simulink library "Linkage"  (R2025b)
settings: Solver=VariableStepAuto  StartTime=0.0  StopTime=10.0  RelTol=1e-3
undefined symbols (not defined in the file): Axle1D, AxleIn, Chassis, Init, RaceFix, RaceSpin, Vehicle, Visual, X, Y, Z
libraries: sm_lib x940, nesl_utility x136, fl_lib x6, Linkage_Systems x2, SteeringWheel x2, Linkage_Decoupled x2, AntiRollBar_Systems x1, Steer_Rack_None x1, Steer_Rack_WheelDrivenRack1UJoint x1
(part 15 of 25)

== system Linkage/Susp/Linkage Decoupled/Steer/Rack Driven Shafts/Driver/Human/Twist ==
  Revolute Joint : sm_lib/Joints/Revolute Joint  Commented=on  JointMode=Normal  CompositeWrenchDir=FollowerOnBase  CompositeWrenchFrame=BaseFrame  SenseConstraintForce=off  SenseConstraintTorque=off  SenseTotalForce=off  SenseTotalTorque=off  PositionTargetSpecify=off  PositionTargetPriority=High  PositionTargetValue=0  PositionTargetValueUnits=deg  VelocityTargetSpecify=off  VelocityTargetPriority=High  VelocityTargetValue=0  VelocityTargetValueUnits=deg/s  EquilibriumPosition=0  EquilibriumPositionUnits=deg  SpringStiffness=dt_k  SpringStiffnessUnits=N*m/deg  DampingCoefficient=dt_b  DampingCoefficientUnits=N*m/(deg/s)  LowerLimitSpecify=off  LowerLimitBound=-90  LowerLimitBoundUnits=deg  LowerLimitStiffness=1e4  LowerLimitStiffnessUnits=N*m/deg  LowerLimitDamping=10  LowerLimitDampingUnits=N*m/(deg/s)  LowerLimitTransitionRegionWidth=0.1  LowerLimitTransitionRegionWidthUnits=deg  UpperLimitSpecify=off  UpperLimitBound=90  UpperLimitBoundUnits=deg  UpperLimitStiffness=1e4  UpperLimitStiffnessUnits=N*m/deg  UpperLimitDamping=10  UpperLimitDampingUnits=N*m/(deg/s)  UpperLimitTransitionRegionWidth=0.1  UpperLimitTransitionRegionWidthUnits=deg  TorqueActuationMode=NoTorque  MotionActuationMode=ComputedMotion  SensePosition=off  SenseVelocity=off  SenseAcceleration=off  SenseTorqueForce=off  SenseLowerLimitTorqueForce=off  SenseUpperLimitTorqueForce=off
  Transform Axis Location B : sm_lib/Frames and Transforms/Rigid Transform  RotationMethod=None  FollAlignAxisA=+X  BaseAlignAxisA=+Y  FollAlignAxisB=+Y  BaseAlignAxisB=+Z  RotationStandardAxis=+Y  RotationAngle=0  RotationAngleUnits=deg  RotationArbitraryAxis=[0 0 1]  RotationSequenceAxes=FollowerAxes  RotationSequence=XYX  RotationSequenceAngles=[0 0 0]  RotationSequenceAnglesUnits=deg  RotationMatrix=[1 0 0; 0 1 0; 0 0 1]  Quaternion=[1 0 0 0]  TranslationMethod=StandardAxis  TranslationCartesianOffset=[0 0 0]  TranslationCartesianOffsetUnits=m  TranslationStandardAxis=-X  TranslationStandardOffset=0.05  TranslationStandardOffsetUnits=m  TranslationROffset=0  TranslationROffsetUnits=m  TranslationThetaOffset=0  TranslationThetaOffsetUnits=deg  TranslationZOffset=0  TranslationZOffsetUnits=m
  Transform Axis Location F : sm_lib/Frames and Transforms/Rigid Transform  RotationMethod=None  FollAlignAxisA=+X  BaseAlignAxisA=+Y  FollAlignAxisB=+Y  BaseAlignAxisB=+Z  RotationStandardAxis=+Y  RotationAngle=0  RotationAngleUnits=deg  RotationArbitraryAxis=[0 0 1]  RotationSequenceAxes=FollowerAxes  RotationSequence=XYX  RotationSequenceAngles=[0 0 0]  RotationSequenceAnglesUnits=deg  RotationMatrix=[1 0 0; 0 1 0; 0 0 1]  Quaternion=[1 0 0 0]  TranslationMethod=StandardAxis  TranslationCartesianOffset=[0 0 0]  TranslationCartesianOffsetUnits=m  TranslationStandardAxis=-X  TranslationStandardOffset=0.05  TranslationStandardOffsetUnits=m  TranslationROffset=0  TranslationROffsetUnits=m  TranslationThetaOffset=0  TranslationThetaOffsetUnits=deg  TranslationZOffset=0  TranslationZOffsetUnits=m
  Transform Axis Orientation B : sm_lib/Frames and Transforms/Rigid Transform  RotationMethod=StandardAxis  FollAlignAxisA=+X  BaseAlignAxisA=+Y  FollAlignAxisB=+Y  BaseAlignAxisB=+Z  RotationStandardAxis=+Y  RotationAngle=120  RotationAngleUnits=deg  RotationArbitraryAxis=[0 0 1]  RotationSequenceAxes=FollowerAxes  RotationSequence=XYX  RotationSequenceAngles=[0 0 0]  RotationSequenceAnglesUnits=deg  RotationMatrix=[1 0 0; 0 1 0; 0 0 1]  Quaternion=[1 0 0 0]  TranslationMethod=None  TranslationCartesianOffset=[0 0 0]  TranslationCartesianOffsetUnits=m  TranslationStandardAxis=+Z  TranslationStandardOffset=0  TranslationStandardOffsetUnits=m  TranslationROffset=0  TranslationROffsetUnits=m  TranslationThetaOffset=0  TranslationThetaOffsetUnits=deg  TranslationZOffset=0  TranslationZOffsetUnits=m
  Transform Axis Orientation F : sm_lib/Frames and Transforms/Rigid Transform  RotationMethod=StandardAxis  FollAlignAxisA=+X  BaseAlignAxisA=+Y  FollAlignAxisB=+Y  BaseAlignAxisB=+Z  RotationStandardAxis=+Y  RotationAngle=120  RotationAngleUnits=deg  RotationArbitraryAxis=[0 0 1]  RotationSequenceAxes=FollowerAxes  RotationSequence=XYX  RotationSequenceAngles=[0 0 0]  RotationSequenceAnglesUnits=deg  RotationMatrix=[1 0 0; 0 1 0; 0 0 1]  Quaternion=[1 0 0 0]  TranslationMethod=None  TranslationCartesianOffset=[0 0 0]  TranslationCartesianOffsetUnits=m  TranslationStandardAxis=+Z  TranslationStandardOffset=0  TranslationStandardOffsetUnits=m  TranslationROffset=0  TranslationROffsetUnits=m  TranslationThetaOffset=0  TranslationThetaOffsetUnits=deg  TranslationZOffset=0  TranslationZOffsetUnits=m
  Transform Universal B : sm_lib/Frames and Transforms/Rigid Transform  RotationMethod=StandardAxis  FollAlignAxisA=+X  BaseAlignAxisA=+Y  FollAlignAxisB=+Y  BaseAlignAxisB=+Z  RotationStandardAxis=+Y  RotationAngle=90  RotationAngleUnits=deg  RotationArbitraryAxis=[0 0 1]  RotationSequenceAxes=FollowerAxes  RotationSequence=XYX  RotationSequenceAngles=[0 0 0]  RotationSequenceAnglesUnits=deg  RotationMatrix=[1 0 0; 0 1 0; 0 0 1]  Quaternion=[1 0 0 0]  TranslationMethod=None  TranslationCartesianOffset=[0 0 0]  TranslationCartesianOffsetUnits=m  TranslationStandardAxis=+Z  TranslationStandardOffset=0  TranslationStandardOffsetUnits=m  TranslationROffset=0  TranslationROffsetUnits=m  TranslationThetaOffset=0  TranslationThetaOffsetUnits=deg  TranslationZOffset=0  TranslationZOffsetUnits=m
  Transform Universal F : sm_lib/Frames and Transforms/Rigid Transform  RotationMethod=StandardAxis  FollAlignAxisA=+X  BaseAlignAxisA=+Y  FollAlignAxisB=+Y  BaseAlignAxisB=+Z  RotationStandardAxis=+Y  RotationAngle=90  RotationAngleUnits=deg  RotationArbitraryAxis=[0 0 1]  RotationSequenceAxes=FollowerAxes  RotationSequence=XYX  RotationSequenceAngles=[0 0 0]  RotationSequenceAnglesUnits=deg  RotationMatrix=[1 0 0; 0 1 0; 0 0 1]  Quaternion=[1 0 0 0]  TranslationMethod=None  TranslationCartesianOffset=[0 0 0]  TranslationCartesianOffsetUnits=m  TranslationStandardAxis=+Z  TranslationStandardOffset=0  TranslationStandardOffsetUnits=m  TranslationROffset=0  TranslationROffsetUnits=m  TranslationThetaOffset=0  TranslationThetaOffsetUnits=deg  TranslationZOffset=0  TranslationZOffsetUnits=m
  Universal Torso : sm_lib/Joints/Universal Joint  JointMode=Normal  CompositeWrenchDir=FollowerOnBase  CompositeWrenchFrame=BaseFrame  SenseConstraintForce=off  SenseConstraintTorque=off  SenseTotalForce=off  SenseTotalTorque=off  RxPositionTargetSpecify=off  RxPositionTargetPriority=High  RxPositionTargetValue=0  RxPositionTargetValueUnits=deg  RxVelocityTargetSpecify=off  RxVelocityTargetPriority=High  RxVelocityTargetValue=0  RxVelocityTargetValueUnits=deg/s  RxEquilibriumPosition=0  RxEquilibriumPositionUnits=deg  RxSpringStiffness=10  RxSpringStiffnessUnits=N*m/deg  RxDampingCoefficient=1  RxDampingCoefficientUnits=N*m/(deg/s)  RxLowerLimitSpecify=off  RxLowerLimitBound=-90  RxLowerLimitBoundUnits=deg  RxLowerLimitStiffness=1e4  RxLowerLimitStiffnessUnits=N*m/deg  RxLowerLimitDamping=10  RxLowerLimitDampingUnits=N*m/(deg/s)  RxLowerLimitTransitionRegionWidth=0.1  RxLowerLimitTransitionRegionWidthUnits=deg  RxUpperLimitSpecify=off  RxUpperLimitBound=90  RxUpperLimitBoundUnits=deg  RxUpperLimitStiffness=1e4  RxUpperLimitStiffnessUnits=N*m/deg  RxUpperLimitDamping=10  RxUpperLimitDampingUnits=N*m/(deg/s)  RxUpperLimitTransitionRegionWidth=0.1  RxUpperLimitTransitionRegionWidthUnits=deg  RxTorqueActuationMode=NoTorque  RxMotionActuationMode=ComputedMotion  RxSensePosition=off  RxSenseVelocity=off  RxSenseAcceleration=off  RxSenseTorqueForce=off  RxSenseLowerLimitTorqueForce=off  RxSenseUpperLimitTorqueForce=off  RyPositionTargetSpecify=off  RyPositionTargetPriority=High  RyPositionTargetValue=0  RyPositionTargetValueUnits=deg  RyVelocityTargetSpecify=off  RyVelocityTargetPriority=High  RyVelocityTargetValue=0  RyVelocityTargetValueUnits=deg/s  RyEquilibriumPosition=0  RyEquilibriumPositionUnits=deg  RySpringStiffness=10  RySpringStiffnessUnits=N*m/deg  RyDampingCoefficient=1  RyDampingCoefficientUnits=N*m/(deg/s)  RyLowerLimitSpecify=off  RyLowerLimitBound=-90  RyLowerLimitBoundUnits=deg  RyLowerLimitStiffness=1e4  RyLowerLimitStiffnessUnits=N*m/deg  RyLowerLimitDamping=10  RyLowerLimitDampingUnits=N*m/(deg/s)  RyLowerLimitTransitionRegionWidth=0.1  RyLowerLimitTransitionRegionWidthUnits=deg  RyUpperLimitSpecify=off  RyUpperLimitBound=90  RyUpperLimitBoundUnits=deg  RyUpperLimitStiffness=1e4  RyUpperLimitStiffnessUnits=N*m/deg  RyUpperLimitDamping=10  RyUpperLimitDampingUnits=N*m/(deg/s)  RyUpperLimitTransitionRegionWidth=0.1  RyUpperLimitTransitionRegionWidthUnits=deg  RyTorqueActuationMode=NoTorque  RyMotionActuationMode=ComputedMotion  RySensePosition=off  RySenseVelocity=off  RySenseAcceleration=off  RySenseTorqueForce=off  RySenseLowerLimitTorqueForce=off  RySenseUpperLimitTorqueForce=off
  T : PMIOPort  Side=Right
  B : PMIOPort  Port=2  Side=Left
  connections:
  Transform Axis Orientation B/RConn1 -- Transform Axis Location B/LConn1
  B/RConn1 -- Transform Axis Orientation B/LConn1
  Transform Axis Orientation F/RConn1 -- Transform Axis Location F/LConn1
  Transform Axis Location B/RConn1 -- Transform Universal B/LConn1
  Transform Axis Orientation F/LConn1 -- T/RConn1
  Transform Axis Location F/RConn1 -- Transform Universal F/LConn1
  Universal Torso/LConn1 -- Transform Universal B/RConn1
  Universal Torso/RConn1 -- Transform Universal F/RConn1

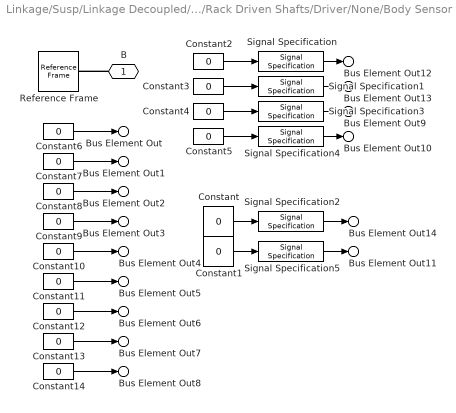
== system Linkage/Susp/Linkage Decoupled/Steer/Rack Driven Shafts/Driver/None/Body Sensor Empty ==
  Constant{,1..14} (15 alike) : Constant  Value=0
  Reference Frame : sm_lib/Frames and Transforms/Reference Frame
  Signal Specification : SignalSpecification  Unit=rad
  Signal Specification1 : SignalSpecification  Unit=rad
  Signal Specification2 : SignalSpecification  Unit=rad
  Signal Specification3 : SignalSpecification  Unit=rad/s
  Signal Specification4 : SignalSpecification  Unit=rad/s
  Signal Specification5 : SignalSpecification  Unit=rad/s
  B : PMIOPort  Side=Left
  Bus Element Out : Outport  VectorParamsAs1DForOutWhenUnconnected=off  PortName=Body  Element=x
  Bus Element Out1 : Outport  VectorParamsAs1DForOutWhenUnconnected=off  PortName=Body  Element=y
  Bus Element Out2 : Outport  VectorParamsAs1DForOutWhenUnconnected=off  PortName=Body  Element=z
  Bus Element Out3 : Outport  VectorParamsAs1DForOutWhenUnconnected=off  PortName=Body  Element=vx
  Bus Element Out4 : Outport  VectorParamsAs1DForOutWhenUnconnected=off  PortName=Body  Element=vy
  Bus Element Out5 : Outport  VectorParamsAs1DForOutWhenUnconnected=off  PortName=Body  Element=vz
  Bus Element Out6 : Outport  VectorParamsAs1DForOutWhenUnconnected=off  PortName=Body  Element=gx
  Bus Element Out7 : Outport  VectorParamsAs1DForOutWhenUnconnected=off  PortName=Body  Element=gy
  Bus Element Out8 : Outport  VectorParamsAs1DForOutWhenUnconnected=off  PortName=Body  Element=gz
  Bus Element Out9 : Outport  VectorParamsAs1DForOutWhenUnconnected=off  PortName=Body  Element=nRoll
  Bus Element Out10 : Outport  VectorParamsAs1DForOutWhenUnconnected=off  PortName=Body  Element=nPitch
  Bus Element Out11 : Outport  VectorParamsAs1DForOutWhenUnconnected=off  PortName=Body  Element=nYaw
  Bus Element Out12 : Outport  VectorParamsAs1DForOutWhenUnconnected=off  PortName=Body  Element=aRoll
  Bus Element Out13 : Outport  VectorParamsAs1DForOutWhenUnconnected=off  PortName=Body  Element=aPitch
  Bus Element Out14 : Outport  VectorParamsAs1DForOutWhenUnconnected=off  PortName=Body  Element=aYaw
  wires:
  Constant14/1 -> Bus Element Out8/1
  Constant11/1 -> Bus Element Out5/1
  Constant12/1 -> Bus Element Out6/1
  Constant7/1 -> Bus Element Out1/1
  Constant13/1 -> Bus Element Out7/1
  Constant10/1 -> Bus Element Out4/1
  Constant8/1 -> Bus Element Out2/1
  Constant6/1 -> Bus Element Out/1
  Constant9/1 -> Bus Element Out3/1
  Signal Specification/1 -> Bus Element Out12/1
  Signal Specification1/1 -> Bus Element Out13/1
  Signal Specification2/1 -> Bus Element Out14/1
  Signal Specification3/1 -> Bus Element Out9/1
  Signal Specification4/1 -> Bus Element Out10/1
  Signal Specification5/1 -> Bus Element Out11/1
  Constant/1 -> Signal Specification2/1
  Constant1/1 -> Signal Specification5/1
  Constant4/1 -> Signal Specification3/1
  Constant5/1 -> Signal Specification4/1
  Constant3/1 -> Signal Specification1/1
  Constant2/1 -> Signal Specification/1
  connections:
  B/RConn1 -- Reference Frame/RConn1

== system Linkage/Susp/Linkage Decoupled/Steer/Rack Driven Shafts/Wheel/FSAE/Transform Steer Axis ==
  Rigid Transform1 : sm_lib/Frames and Transforms/Rigid Transform  RotationMethod=None  FollAlignAxisA=+X  BaseAlignAxisA=+Y  FollAlignAxisB=+Y  BaseAlignAxisB=+Z  RotationStandardAxis=+Z  RotationAngle=0.0  RotationAngleUnits=deg  RotationArbitraryAxis=[0 0 1]  RotationSequenceAxes=FollowerAxes  RotationSequence=XYX  RotationSequenceAngles=[0 0 0]  RotationSequenceAnglesUnits=deg  RotationMatrix=[1 0 0; 0 1 0; 0 0 1]  Quaternion=[1 0 0 0]  TranslationMethod=Cartesian  TranslationCartesianOffset=[0 -0.4664 -0.3791]  TranslationCartesianOffsetUnits=m  TranslationStandardAxis=+Z  TranslationStandardOffset=0  TranslationStandardOffsetUnits=m  TranslationROffset=0  TranslationROffsetUnits=m  TranslationThetaOffset=0  TranslationThetaOffsetUnits=deg  TranslationZOffset=0  TranslationZOffsetUnits=m
  Rigid Transform2 : sm_lib/Frames and Transforms/Rigid Transform  RotationMethod=RotationMatrix  FollAlignAxisA=+X  BaseAlignAxisA=+Y  FollAlignAxisB=+Y  BaseAlignAxisB=+Z  RotationStandardAxis=+Z  RotationAngle=0.0  RotationAngleUnits=deg  RotationArbitraryAxis=[0 0 1]  RotationSequenceAxes=FollowerAxes  RotationSequence=XYX  RotationSequenceAngles=[0 0 0]  RotationSequenceAnglesUnits=deg  RotationMatrix=[0.5 0.866 -6.661e-16; -0.8602 0.4967 0.1153; 0.09988 -0.05766 0.9933]  Quaternion=[1 0 0 0]  TranslationMethod=None  TranslationCartesianOffset=[0 0 0]  TranslationCartesianOffsetUnits=m  TranslationStandardAxis=+Z  TranslationStandardOffset=0  TranslationStandardOffsetUnits=m  TranslationROffset=0  TranslationROffsetUnits=m  TranslationThetaOffset=0  TranslationThetaOffsetUnits=deg  TranslationZOffset=0  TranslationZOffsetUnits=m
  Rigid Transform4 : sm_lib/Frames and Transforms/Rigid Transform  RotationMethod=StandardAxis  FollAlignAxisA=+X  BaseAlignAxisA=+Y  FollAlignAxisB=+Y  BaseAlignAxisB=+Z  RotationStandardAxis=+Z  RotationAngle=150  RotationAngleUnits=deg  RotationArbitraryAxis=[0 0 1]  RotationSequenceAxes=FollowerAxes  RotationSequence=XYX  RotationSequenceAngles=[0 0 0]  RotationSequenceAnglesUnits=deg  RotationMatrix=[1 0 0; 0 1 0; 0 0 1]  Quaternion=[1 0 0 0]  TranslationMethod=StandardAxis  TranslationCartesianOffset=[0 0 0]  TranslationCartesianOffsetUnits=m  TranslationStandardAxis=+Z  TranslationStandardOffset=0.09  TranslationStandardOffsetUnits=m  TranslationROffset=0  TranslationROffsetUnits=m  TranslationThetaOffset=0  TranslationThetaOffsetUnits=deg  TranslationZOffset=0  TranslationZOffsetUnits=m
  F : PMIOPort  Side=Left
  B : PMIOPort  Port=2  Side=Right
  connections:
  Rigid Transform2/RConn1 -- Rigid Transform4/LConn1
  F/RConn1 -- Rigid Transform4/RConn1
  Rigid Transform1/LConn1 -- Rigid Transform2/LConn1
  B/RConn1 -- Rigid Transform1/RConn1

== system Linkage/Susp/Linkage Decoupled/Steer/Rack Static Shafts/Driver/Human/Arm L ==
  Arm Lower L : Subsystem
  Arm Upper L : Subsystem
  Hand L : Subsystem
  Revolute ElbowL : sm_lib/Joints/Revolute Joint  JointMode=Normal  CompositeWrenchDir=FollowerOnBase  CompositeWrenchFrame=BaseFrame  SenseConstraintForce=off  SenseConstraintTorque=off  SenseTotalForce=off  SenseTotalTorque=off  PositionTargetSpecify=on  PositionTargetPriority=Low  PositionTargetValue=50  PositionTargetValueUnits=deg  VelocityTargetSpecify=off  VelocityTargetPriority=High  VelocityTargetValue=0  VelocityTargetValueUnits=deg/s  EquilibriumPosition=0  EquilibriumPositionUnits=deg  SpringStiffness=0  SpringStiffnessUnits=N*m/deg  DampingCoefficient=0  DampingCoefficientUnits=N*m/(deg/s)  LowerLimitSpecify=off  LowerLimitBound=-90  LowerLimitBoundUnits=deg  LowerLimitStiffness=1e4  LowerLimitStiffnessUnits=N*m/deg  LowerLimitDamping=10  LowerLimitDampingUnits=N*m/(deg/s)  LowerLimitTransitionRegionWidth=0.1  LowerLimitTransitionRegionWidthUnits=deg  UpperLimitSpecify=off  UpperLimitBound=90  UpperLimitBoundUnits=deg  UpperLimitStiffness=1e4  UpperLimitStiffnessUnits=N*m/deg  UpperLimitDamping=10  UpperLimitDampingUnits=N*m/(deg/s)  UpperLimitTransitionRegionWidth=0.1  UpperLimitTransitionRegionWidthUnits=deg  TorqueActuationMode=NoTorque  MotionActuationMode=ComputedMotion  SensePosition=off  SenseVelocity=off  SenseAcceleration=off  SenseTorqueForce=off  SenseLowerLimitTorqueForce=off  SenseUpperLimitTorqueForce=off
  Spherical ShoulderL : sm_lib/Joints/Spherical Joint  JointMode=Normal  CompositeWrenchDir=FollowerOnBase  CompositeWrenchFrame=BaseFrame  SenseConstraintForce=off  SenseConstraintTorque=off  SenseTotalForce=off  SenseTotalTorque=off  PositionTargetSpecify=off  PositionTargetPriority=High  PositionTargetRotationMethod=None  PositionTargetFollAlignAxisA=+X  PositionTargetBaseAlignAxisA=+Y  PositionTargetFollAlignAxisB=+Y  PositionTargetBaseAlignAxisB=+Z  PositionTargetRotationStandardAxis=+Z  PositionTargetRotationAngle=0.0  PositionTargetRotationAngleUnits=deg  PositionTargetRotationArbitraryAxis=[0 0 1]  PositionTargetRotationSequenceAxes=FollowerAxes  PositionTargetRotationSequence=XYX  PositionTargetRotationSequenceAngles=[0 0 0]  PositionTargetRotationSequenceAnglesUnits=deg  PositionTargetRotationMatrix=[1 0 0; 0 1 0; 0 0 1]  PositionTargetQuaternion=[1 0 0 0]  VelocityTargetSpecify=off  VelocityTargetPriority=High  VelocityTargetValue=[0 0 0]  VelocityTargetValueUnits=deg/s  VelocityTargetInFollowerFrame=on  EqPosRotationMethod=None  EqPosFollAlignAxisA=+X  EqPosBaseAlignAxisA=+Y  EqPosFollAlignAxisB=+Y  EqPosBaseAlignAxisB=+Z  EqPosRotationStandardAxis=+Z  EqPosRotationAngle=0.0  EqPosRotationAngleUnits=deg  EqPosRotationArbitraryAxis=[0 0 1]  EqPosRotationSequenceAxes=FollowerAxes  EqPosRotationSequence=XYX  EqPosRotationSequenceAngles=[0 0 0]  EqPosRotationSequenceAnglesUnits=deg  EqPosRotationMatrix=[1 0 0; 0 1 0; 0 0 1]  EqPosQuaternion=[1 0 0 0]  SpringStiffness=0  SpringStiffnessUnits=N*m/deg  DampingCoefficient=0  DampingCoefficientUnits=N*m/(deg/s)  LowerLimitSpecify=off  LowerLimitBound=15  LowerLimitBoundUnits=deg  LowerLimitStiffness=1e4  LowerLimitStiffnessUnits=N*m/deg  LowerLimitDamping=10  LowerLimitDampingUnits=N*m/(deg/s)  LowerLimitTransitionRegionWidth=0.1  LowerLimitTransitionRegionWidthUnits=deg  UpperLimitSpecify=off  UpperLimitBound=45  UpperLimitBoundUnits=deg  UpperLimitStiffness=1e4  UpperLimitStiffnessUnits=N*m/deg  UpperLimitDamping=10  UpperLimitDampingUnits=N*m/(deg/s)  UpperLimitTransitionRegionWidth=0.1  UpperLimitTransitionRegionWidthUnits=deg  TorqueActuationMode=NoTorque  ActuateTorqueX=off  ActuateTorqueY=off  ActuateTorqueZ=off  ActuateTorque=off  ActuationFrame=BaseFrame  SensePosition=off  SenseVelocityX=off  SenseVelocityY=off  SenseVelocityZ=off  SenseVelocity=off  SenseAccelerationX=off  SenseAccelerationY=off  SenseAccelerationZ=off  SenseAcceleration=off  SenseLowerLimitTorqueMag=off  SenseUpperLimitTorqueMag=off  SensingFrame=BaseFrame
  Universal WristL : sm_lib/Joints/Universal Joint  JointMode=Normal  CompositeWrenchDir=FollowerOnBase  CompositeWrenchFrame=BaseFrame  SenseConstraintForce=off  SenseConstraintTorque=off  SenseTotalForce=off  SenseTotalTorque=off  RxPositionTargetSpecify=off  RxPositionTargetPriority=High  RxPositionTargetValue=0  RxPositionTargetValueUnits=deg  RxVelocityTargetSpecify=off  RxVelocityTargetPriority=High  RxVelocityTargetValue=0  RxVelocityTargetValueUnits=deg/s  RxEquilibriumPosition=0  RxEquilibriumPositionUnits=deg  RxSpringStiffness=0  RxSpringStiffnessUnits=N*m/deg  RxDampingCoefficient=0  RxDampingCoefficientUnits=N*m/(deg/s)  RxLowerLimitSpecify=off  RxLowerLimitBound=-90  RxLowerLimitBoundUnits=deg  RxLowerLimitStiffness=1e4  RxLowerLimitStiffnessUnits=N*m/deg  RxLowerLimitDamping=10  RxLowerLimitDampingUnits=N*m/(deg/s)  RxLowerLimitTransitionRegionWidth=0.1  RxLowerLimitTransitionRegionWidthUnits=deg  RxUpperLimitSpecify=off  RxUpperLimitBound=90  RxUpperLimitBoundUnits=deg  RxUpperLimitStiffness=1e4  RxUpperLimitStiffnessUnits=N*m/deg  RxUpperLimitDamping=10  RxUpperLimitDampingUnits=N*m/(deg/s)  RxUpperLimitTransitionRegionWidth=0.1  RxUpperLimitTransitionRegionWidthUnits=deg  RxTorqueActuationMode=NoTorque  RxMotionActuationMode=ComputedMotion  RxSensePosition=off  RxSenseVelocity=off  RxSenseAcceleration=off  RxSenseTorqueForce=off  RxSenseLowerLimitTorqueForce=off  RxSenseUpperLimitTorqueForce=off  RyPositionTargetSpecify=off  RyPositionTargetPriority=High  RyPositionTargetValue=0  RyPositionTargetValueUnits=deg  RyVelocityTargetSpecify=off  RyVelocityTargetPriority=High  RyVelocityTargetValue=0  RyVelocityTargetValueUnits=deg/s  RyEquilibriumPosition=0  RyEquilibriumPositionUnits=deg  RySpringStiffness=0  RySpringStiffnessUnits=N*m/deg  RyDampingCoefficient=0  RyDampingCoefficientUnits=N*m/(deg/s)  RyLowerLimitSpecify=off  RyLowerLimitBound=-90  RyLowerLimitBoundUnits=deg  RyLowerLimitStiffness=1e4  RyLowerLimitStiffnessUnits=N*m/deg  RyLowerLimitDamping=10  RyLowerLimitDampingUnits=N*m/(deg/s)  RyLowerLimitTransitionRegionWidth=0.1  RyLowerLimitTransitionRegionWidthUnits=deg  RyUpperLimitSpecify=off  RyUpperLimitBound=90  RyUpperLimitBoundUnits=deg  RyUpperLimitStiffness=1e4  RyUpperLimitStiffnessUnits=N*m/deg  RyUpperLimitDamping=10  RyUpperLimitDampingUnits=N*m/(deg/s)  RyUpperLimitTransitionRegionWidth=0.1  RyUpperLimitTransitionRegionWidthUnits=deg  RyTorqueActuationMode=NoTorque  RyMotionActuationMode=ComputedMotion  RySensePosition=off  RySenseVelocity=off  RySenseAcceleration=off  RySenseTorqueForce=off  RySenseLowerLimitTorqueForce=off  RySenseUpperLimitTorqueForce=off
  Sh : PMIOPort  Side=Left
  Grip : PMIOPort  Port=2  Side=Right
  connections:
  Spherical ShoulderL/LConn1 -- Sh/RConn1
  Arm Lower L/RConn1 -- Universal WristL/LConn1
  Arm Lower L/LConn1 -- Revolute ElbowL/RConn1
  Hand L/RConn1 -- Grip/RConn1
  Universal WristL/RConn1 -- Hand L/LConn1
  Spherical ShoulderL/RConn1 -- Arm Upper L/LConn1
  Revolute ElbowL/LConn1 -- Arm Upper L/RConn1

== system Linkage/Susp/Linkage Decoupled/Steer/Rack Static Shafts/Driver/Human/Arm R ==
  Arm Lower R : Subsystem
  Arm Upper R : Subsystem
  Hand R : Subsystem
  Revolute ElbowR : sm_lib/Joints/Revolute Joint  JointMode=Normal  CompositeWrenchDir=FollowerOnBase  CompositeWrenchFrame=BaseFrame  SenseConstraintForce=off  SenseConstraintTorque=off  SenseTotalForce=off  SenseTotalTorque=off  PositionTargetSpecify=on  PositionTargetPriority=Low  PositionTargetValue=50  PositionTargetValueUnits=deg  VelocityTargetSpecify=off  VelocityTargetPriority=High  VelocityTargetValue=0  VelocityTargetValueUnits=deg/s  EquilibriumPosition=0  EquilibriumPositionUnits=deg  SpringStiffness=0  SpringStiffnessUnits=N*m/deg  DampingCoefficient=0  DampingCoefficientUnits=N*m/(deg/s)  LowerLimitSpecify=off  LowerLimitBound=-90  LowerLimitBoundUnits=deg  LowerLimitStiffness=1e4  LowerLimitStiffnessUnits=N*m/deg  LowerLimitDamping=10  LowerLimitDampingUnits=N*m/(deg/s)  LowerLimitTransitionRegionWidth=0.1  LowerLimitTransitionRegionWidthUnits=deg  UpperLimitSpecify=off  UpperLimitBound=90  UpperLimitBoundUnits=deg  UpperLimitStiffness=1e4  UpperLimitStiffnessUnits=N*m/deg  UpperLimitDamping=10  UpperLimitDampingUnits=N*m/(deg/s)  UpperLimitTransitionRegionWidth=0.1  UpperLimitTransitionRegionWidthUnits=deg  TorqueActuationMode=NoTorque  MotionActuationMode=ComputedMotion  SensePosition=off  SenseVelocity=off  SenseAcceleration=off  SenseTorqueForce=off  SenseLowerLimitTorqueForce=off  SenseUpperLimitTorqueForce=off
  Spherical ShoulderR : sm_lib/Joints/Spherical Joint  JointMode=Normal  CompositeWrenchDir=FollowerOnBase  CompositeWrenchFrame=BaseFrame  SenseConstraintForce=off  SenseConstraintTorque=off  SenseTotalForce=off  SenseTotalTorque=off  PositionTargetSpecify=off  PositionTargetPriority=High  PositionTargetRotationMethod=None  PositionTargetFollAlignAxisA=+X  PositionTargetBaseAlignAxisA=+Y  PositionTargetFollAlignAxisB=+Y  PositionTargetBaseAlignAxisB=+Z  PositionTargetRotationStandardAxis=+Z  PositionTargetRotationAngle=0.0  PositionTargetRotationAngleUnits=deg  PositionTargetRotationArbitraryAxis=[0 0 1]  PositionTargetRotationSequenceAxes=FollowerAxes  PositionTargetRotationSequence=XYX  PositionTargetRotationSequenceAngles=[0 0 0]  PositionTargetRotationSequenceAnglesUnits=deg  PositionTargetRotationMatrix=[1 0 0; 0 1 0; 0 0 1]  PositionTargetQuaternion=[1 0 0 0]  VelocityTargetSpecify=off  VelocityTargetPriority=High  VelocityTargetValue=[0 0 0]  VelocityTargetValueUnits=deg/s  VelocityTargetInFollowerFrame=on  EqPosRotationMethod=None  EqPosFollAlignAxisA=+X  EqPosBaseAlignAxisA=+Y  EqPosFollAlignAxisB=+Y  EqPosBaseAlignAxisB=+Z  EqPosRotationStandardAxis=+Z  EqPosRotationAngle=0.0  EqPosRotationAngleUnits=deg  EqPosRotationArbitraryAxis=[0 0 1]  EqPosRotationSequenceAxes=FollowerAxes  EqPosRotationSequence=XYX  EqPosRotationSequenceAngles=[0 0 0]  EqPosRotationSequenceAnglesUnits=deg  EqPosRotationMatrix=[1 0 0; 0 1 0; 0 0 1]  EqPosQuaternion=[1 0 0 0]  SpringStiffness=0  SpringStiffnessUnits=N*m/deg  DampingCoefficient=0  DampingCoefficientUnits=N*m/(deg/s)  LowerLimitSpecify=off  LowerLimitBound=15  LowerLimitBoundUnits=deg  LowerLimitStiffness=1e4  LowerLimitStiffnessUnits=N*m/deg  LowerLimitDamping=10  LowerLimitDampingUnits=N*m/(deg/s)  LowerLimitTransitionRegionWidth=0.1  LowerLimitTransitionRegionWidthUnits=deg  UpperLimitSpecify=off  UpperLimitBound=45  UpperLimitBoundUnits=deg  UpperLimitStiffness=1e4  UpperLimitStiffnessUnits=N*m/deg  UpperLimitDamping=10  UpperLimitDampingUnits=N*m/(deg/s)  UpperLimitTransitionRegionWidth=0.1  UpperLimitTransitionRegionWidthUnits=deg  TorqueActuationMode=NoTorque  ActuateTorqueX=off  ActuateTorqueY=off  ActuateTorqueZ=off  ActuateTorque=off  ActuationFrame=BaseFrame  SensePosition=off  SenseVelocityX=off  SenseVelocityY=off  SenseVelocityZ=off  SenseVelocity=off  SenseAccelerationX=off  SenseAccelerationY=off  SenseAccelerationZ=off  SenseAcceleration=off  SenseLowerLimitTorqueMag=off  SenseUpperLimitTorqueMag=off  SensingFrame=BaseFrame
  Universal WristR : sm_lib/Joints/Universal Joint  JointMode=Normal  CompositeWrenchDir=FollowerOnBase  CompositeWrenchFrame=BaseFrame  SenseConstraintForce=off  SenseConstraintTorque=off  SenseTotalForce=off  SenseTotalTorque=off  RxPositionTargetSpecify=off  RxPositionTargetPriority=High  RxPositionTargetValue=0  RxPositionTargetValueUnits=deg  RxVelocityTargetSpecify=off  RxVelocityTargetPriority=High  RxVelocityTargetValue=0  RxVelocityTargetValueUnits=deg/s  RxEquilibriumPosition=0  RxEquilibriumPositionUnits=deg  RxSpringStiffness=0  RxSpringStiffnessUnits=N*m/deg  RxDampingCoefficient=0  RxDampingCoefficientUnits=N*m/(deg/s)  RxLowerLimitSpecify=off  RxLowerLimitBound=-90  RxLowerLimitBoundUnits=deg  RxLowerLimitStiffness=1e4  RxLowerLimitStiffnessUnits=N*m/deg  RxLowerLimitDamping=10  RxLowerLimitDampingUnits=N*m/(deg/s)  RxLowerLimitTransitionRegionWidth=0.1  RxLowerLimitTransitionRegionWidthUnits=deg  RxUpperLimitSpecify=off  RxUpperLimitBound=90  RxUpperLimitBoundUnits=deg  RxUpperLimitStiffness=1e4  RxUpperLimitStiffnessUnits=N*m/deg  RxUpperLimitDamping=10  RxUpperLimitDampingUnits=N*m/(deg/s)  RxUpperLimitTransitionRegionWidth=0.1  RxUpperLimitTransitionRegionWidthUnits=deg  RxTorqueActuationMode=NoTorque  RxMotionActuationMode=ComputedMotion  RxSensePosition=off  RxSenseVelocity=off  RxSenseAcceleration=off  RxSenseTorqueForce=off  RxSenseLowerLimitTorqueForce=off  RxSenseUpperLimitTorqueForce=off  RyPositionTargetSpecify=off  RyPositionTargetPriority=High  RyPositionTargetValue=0  RyPositionTargetValueUnits=deg  RyVelocityTargetSpecify=off  RyVelocityTargetPriority=High  RyVelocityTargetValue=0  RyVelocityTargetValueUnits=deg/s  RyEquilibriumPosition=0  RyEquilibriumPositionUnits=deg  RySpringStiffness=0  RySpringStiffnessUnits=N*m/deg  RyDampingCoefficient=0  RyDampingCoefficientUnits=N*m/(deg/s)  RyLowerLimitSpecify=off  RyLowerLimitBound=-90  RyLowerLimitBoundUnits=deg  RyLowerLimitStiffness=1e4  RyLowerLimitStiffnessUnits=N*m/deg  RyLowerLimitDamping=10  RyLowerLimitDampingUnits=N*m/(deg/s)  RyLowerLimitTransitionRegionWidth=0.1  RyLowerLimitTransitionRegionWidthUnits=deg  RyUpperLimitSpecify=off  RyUpperLimitBound=90  RyUpperLimitBoundUnits=deg  RyUpperLimitStiffness=1e4  RyUpperLimitStiffnessUnits=N*m/deg  RyUpperLimitDamping=10  RyUpperLimitDampingUnits=N*m/(deg/s)  RyUpperLimitTransitionRegionWidth=0.1  RyUpperLimitTransitionRegionWidthUnits=deg  RyTorqueActuationMode=NoTorque  RyMotionActuationMode=ComputedMotion  RySensePosition=off  RySenseVelocity=off  RySenseAcceleration=off  RySenseTorqueForce=off  RySenseLowerLimitTorqueForce=off  RySenseUpperLimitTorqueForce=off
  Grip : PMIOPort  Side=Right
  Sh : PMIOPort  Port=2  Side=Left
  connections:
  Hand R/RConn1 -- Grip/RConn1
  Arm Upper R/RConn1 -- Revolute ElbowR/LConn1
  Revolute ElbowR/RConn1 -- Arm Lower R/LConn1
  Universal WristR/RConn1 -- Hand R/LConn1
  Arm Upper R/LConn1 -- Spherical ShoulderR/RConn1
  Arm Lower R/RConn1 -- Universal WristR/LConn1
  Sh/RConn1 -- Spherical ShoulderR/LConn1

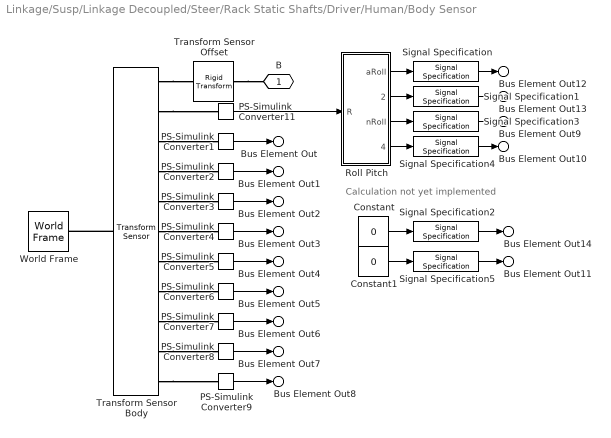
== system Linkage/Susp/Linkage Decoupled/Steer/Rack Static Shafts/Driver/Human/Body Sensor ==
  note: Calculation not yet implemented
  Constant : Constant  Value=0
  Constant1 : Constant  Value=0
  PS-Simulink Converter1 : nesl_utility/PS-Simulink Converter  PhysicalDomain=network_engine_domain  SubClassName=ps_output  LeftPortType=input  RightPortType=output  PseudoPeriodic=off  Frequencies=[]  VectorFormat=1-D array  Unit=m  AffineConversion=off
  PS-Simulink Converter11 : nesl_utility/PS-Simulink Converter  PhysicalDomain=network_engine_domain  SubClassName=ps_output  LeftPortType=input  RightPortType=output  PseudoPeriodic=off  Frequencies=[]  VectorFormat=1-D array  Unit=1  AffineConversion=off
  PS-Simulink Converter2 : nesl_utility/PS-Simulink Converter  PhysicalDomain=network_engine_domain  SubClassName=ps_output  LeftPortType=input  RightPortType=output  PseudoPeriodic=off  Frequencies=[]  VectorFormat=1-D array  Unit=m  AffineConversion=off
  PS-Simulink Converter3 : nesl_utility/PS-Simulink Converter  PhysicalDomain=network_engine_domain  SubClassName=ps_output  LeftPortType=input  RightPortType=output  PseudoPeriodic=off  Frequencies=[]  VectorFormat=1-D array  Unit=m  AffineConversion=off
  PS-Simulink Converter4 : nesl_utility/PS-Simulink Converter  PhysicalDomain=network_engine_domain  SubClassName=ps_output  LeftPortType=input  RightPortType=output  PseudoPeriodic=off  Frequencies=[]  VectorFormat=1-D array  Unit=m/s  AffineConversion=off
  PS-Simulink Converter5 : nesl_utility/PS-Simulink Converter  PhysicalDomain=network_engine_domain  SubClassName=ps_output  LeftPortType=input  RightPortType=output  PseudoPeriodic=off  Frequencies=[]  VectorFormat=1-D array  Unit=m/s  AffineConversion=off
  PS-Simulink Converter6 : nesl_utility/PS-Simulink Converter  PhysicalDomain=network_engine_domain  SubClassName=ps_output  LeftPortType=input  RightPortType=output  PseudoPeriodic=off  Frequencies=[]  VectorFormat=1-D array  Unit=m/s  AffineConversion=off
  PS-Simulink Converter7 : nesl_utility/PS-Simulink Converter  PhysicalDomain=network_engine_domain  SubClassName=ps_output  LeftPortType=input  RightPortType=output  PseudoPeriodic=off  Frequencies=[]  VectorFormat=1-D array  Unit=m/s^2  AffineConversion=off
  PS-Simulink Converter8 : nesl_utility/PS-Simulink Converter  PhysicalDomain=network_engine_domain  SubClassName=ps_output  LeftPortType=input  RightPortType=output  PseudoPeriodic=off  Frequencies=[]  VectorFormat=1-D array  Unit=m/s^2  AffineConversion=off
  PS-Simulink Converter9 : nesl_utility/PS-Simulink Converter  PhysicalDomain=network_engine_domain  SubClassName=ps_output  LeftPortType=input  RightPortType=output  PseudoPeriodic=off  Frequencies=[]  VectorFormat=1-D array  Unit=m/s^2  AffineConversion=off
  Roll Pitch : Subsystem
  Signal Specification : SignalSpecification  Unit=rad
  Signal Specification1 : SignalSpecification  Unit=rad
  Signal Specification2 : SignalSpecification  Unit=rad
  Signal Specification3 : SignalSpecification  Unit=rad/s
  Signal Specification4 : SignalSpecification  Unit=rad/s
  Signal Specification5 : SignalSpecification  Unit=rad/s
  Transform Sensor Offset : sm_lib/Frames and Transforms/Rigid Transform  RotationMethod=None  FollAlignAxisA=+X  BaseAlignAxisA=+Y  FollAlignAxisB=+Y  BaseAlignAxisB=+Z  RotationStandardAxis=+Z  RotationAngle=0.0  RotationAngleUnits=deg  RotationArbitraryAxis=[0 0 1]  RotationSequenceAxes=FollowerAxes  RotationSequence=XYX  RotationSequenceAngles=[0 0 0]  RotationSequenceAnglesUnits=deg  RotationMatrix=[1 0 0; 0 1 0; 0 0 1]  Quaternion=[1 0 0 0]  TranslationMethod=Cartesian  TranslationCartesianOffset=offset_body_sensor  TranslationCartesianOffsetUnits=m  TranslationStandardAxis=+Z  TranslationStandardOffset=0  TranslationStandardOffsetUnits=m  TranslationROffset=0  TranslationROffsetUnits=m  TranslationThetaOffset=0  TranslationThetaOffsetUnits=deg  TranslationZOffset=0  TranslationZOffsetUnits=m
  Transform Sensor Body : sm_lib/Frames and Transforms/Transform Sensor  MeasurementFrame=NonRotatingFollower  RotationSequence=XYX  SenseAngle=off  SenseAxis=off  SenseQ=off  SenseR=on  SenseRotationSequence=off  SenseOmegaX=off  SenseOmegaY=off  SenseOmegaZ=off  SenseOmega=off  SenseQDot=off  SenseRDot=off  SenseRotationSequenceDot=off  SenseAlphaX=off  SenseAlphaY=off  SenseAlphaZ=off  SenseAlpha=off  SenseQDDot=off  SenseRDDot=off  SenseX=on  SenseY=on  SenseZ=on  SenseXYZ=off  SenseRad=off  SenseAzim=off  SenseDist=off  SenseInc=off  SenseXDot=on  SenseYDot=on  SenseZDot=on  SenseXYZDot=off  SenseRadDot=off  SenseAzimDot=off  SenseDistDot=off  SenseIncDot=off  SenseXDDot=on  SenseYDDot=on  SenseZDDot=on  SenseXYZDDot=off  SenseRadDDot=off  SenseAzimDDot=off  SenseDistDDot=off  SenseIncDDot=off
  World Frame : sm_lib/Frames and Transforms/World Frame
  B : PMIOPort  Side=Left
  Bus Element Out : Outport  VectorParamsAs1DForOutWhenUnconnected=off  PortName=Body  Element=x
  Bus Element Out1 : Outport  VectorParamsAs1DForOutWhenUnconnected=off  PortName=Body  Element=y
  Bus Element Out2 : Outport  VectorParamsAs1DForOutWhenUnconnected=off  PortName=Body  Element=z
  Bus Element Out3 : Outport  VectorParamsAs1DForOutWhenUnconnected=off  PortName=Body  Element=vx
  Bus Element Out4 : Outport  VectorParamsAs1DForOutWhenUnconnected=off  PortName=Body  Element=vy
  Bus Element Out5 : Outport  VectorParamsAs1DForOutWhenUnconnected=off  PortName=Body  Element=vz
  Bus Element Out6 : Outport  VectorParamsAs1DForOutWhenUnconnected=off  PortName=Body  Element=gx
  Bus Element Out7 : Outport  VectorParamsAs1DForOutWhenUnconnected=off  PortName=Body  Element=gy
  Bus Element Out8 : Outport  VectorParamsAs1DForOutWhenUnconnected=off  PortName=Body  Element=gz
  Bus Element Out9 : Outport  VectorParamsAs1DForOutWhenUnconnected=off  PortName=Body  Element=nRoll
  Bus Element Out10 : Outport  VectorParamsAs1DForOutWhenUnconnected=off  PortName=Body  Element=nPitch
  Bus Element Out11 : Outport  VectorParamsAs1DForOutWhenUnconnected=off  PortName=Body  Element=nYaw
  Bus Element Out12 : Outport  VectorParamsAs1DForOutWhenUnconnected=off  PortName=Body  Element=aRoll
  Bus Element Out13 : Outport  VectorParamsAs1DForOutWhenUnconnected=off  PortName=Body  Element=aPitch
  Bus Element Out14 : Outport  VectorParamsAs1DForOutWhenUnconnected=off  PortName=Body  Element=aYaw
  wires:
  Roll Pitch/1(aRoll) -> Signal Specification/1
  Roll Pitch/2(aPitch) -> Signal Specification1/1
  Roll Pitch/4(nPitch) -> Signal Specification4/1
  Roll Pitch/3(nRoll) -> Signal Specification3/1
  Constant1/1 -> Signal Specification5/1
  Constant/1 -> Signal Specification2/1
  Signal Specification5/1 -> Bus Element Out11/1
  Signal Specification4/1 -> Bus Element Out10/1
  Signal Specification3/1 -> Bus Element Out9/1
  Signal Specification2/1 -> Bus Element Out14/1
  Signal Specification1/1 -> Bus Element Out13/1
  Signal Specification/1 -> Bus Element Out12/1
  PS-Simulink Converter4/1 -> Bus Element Out3/1
  PS-Simulink Converter1/1 -> Bus Element Out/1
  PS-Simulink Converter3/1 -> Bus Element Out2/1
  PS-Simulink Converter5/1 -> Bus Element Out4/1
  PS-Simulink Converter8/1 -> Bus Element Out7/1
  PS-Simulink Converter2/1 -> Bus Element Out1/1
  PS-Simulink Converter7/1 -> Bus Element Out6/1
  PS-Simulink Converter6/1 -> Bus Element Out5/1
  PS-Simulink Converter11/1 -> Roll Pitch/1(R)
  PS-Simulink Converter9/1 -> Bus Element Out8/1
  connections:
  Transform Sensor Body/RConn1 -- Transform Sensor Offset/RConn1
  Transform Sensor Body/RConn6 -- PS-Simulink Converter4/LConn1
  Transform Sensor Body/RConn8 -- PS-Simulink Converter6/LConn1
  Transform Sensor Body/RConn9 -- PS-Simulink Converter7/LConn1
  Transform Sensor Body/RConn10 -- PS-Simulink Converter8/LConn1
  Transform Sensor Offset/LConn1 -- B/RConn1
  Transform Sensor Body/LConn1 -- World Frame/RConn1
  Transform Sensor Body/RConn3 -- PS-Simulink Converter1/LConn1
  Transform Sensor Body/RConn7 -- PS-Simulink Converter5/LConn1
  Transform Sensor Body/RConn2 -- PS-Simulink Converter11/LConn1
  Transform Sensor Body/RConn11 -- PS-Simulink Converter9/LConn1
  Transform Sensor Body/RConn4 -- PS-Simulink Converter2/LConn1
  Transform Sensor Body/RConn5 -- PS-Simulink Converter3/LConn1

== system Linkage/Susp/Linkage Decoupled/Steer/Rack Static Shafts/Driver/Human/Head ==
  ReferenceFrame : sm_lib/Frames and Transforms/Reference Frame
  Solid : sm_lib/Body Elements/File Solid  ExtGeomFileName=Human_head.STEP  UnitType=FromFile  ExtGeomFileUnits=m  StepReaderType=HEX  ExportConvexHullGeometry=off  InertiaType=CalculateFromGeometry  BasedOnType=Density  Density=rho_human  DensityUnits=kg/m^3  Mass=0  MassUnits=kg  CenterOfMass=[0 0 0]  CenterOfMassUnits=cm  MomentsOfInertia=[1 1 1]  MomentsOfInertiaUnits=kg*cm^2  ProductsOfInertia=[0 0 0]  ProductsOfInertiaUnits=kg*cm^2  GraphicType=FromGeometry  MarkerShape=Sphere  MarkerSize=10  GraphicVisPropType=SimpleVisualProperties  GraphicDiffuseColor=clr_human  GraphicOpacity=opc_human  GraphicSpecularColor=[0.5 0.5 0.5 1.0]  GraphicAmbientColor=[0.15 0.15 0.15 1.0]  GraphicEmissiveColor=[0.0 0.0 0.0 1.0]  GraphicShininess=75  DoExposeReferenceFrame=on  SerializedFrames=<Frames/>
  Transform : sm_lib/Frames and Transforms/Rigid Transform  RotationMethod=ArbitraryAxis  FollAlignAxisA=+X  BaseAlignAxisA=+Y  FollAlignAxisB=+Y  BaseAlignAxisB=+Z  RotationStandardAxis=+Z  RotationAngle=2.0943951023932  RotationAngleUnits=rad  RotationArbitraryAxis=[0.577350269189626 0.577350269189626 0.577350269189626]  RotationSequenceAxes=FollowerAxes  RotationSequence=XYX  RotationSequenceAngles=[0 0 0]  RotationSequenceAnglesUnits=deg  RotationMatrix=[1 0 0; 0 1 0; 0 0 1]  Quaternion=[1 0 0 0]  TranslationMethod=Cartesian  TranslationCartesianOffset=[5.00894645716943e-14 20.8274781700019 499.860076899999]  TranslationCartesianOffsetUnits=mm  TranslationStandardAxis=+Z  TranslationStandardOffset=0  TranslationStandardOffsetUnits=mm  TranslationROffset=0  TranslationROffsetUnits=m  TranslationThetaOffset=0  TranslationThetaOffsetUnits=deg  TranslationZOffset=0  TranslationZOffsetUnits=m
  Transform Head Center : sm_lib/Frames and Transforms/Rigid Transform  RotationMethod=StandardAxis  FollAlignAxisA=+X  BaseAlignAxisA=+Y  FollAlignAxisB=+Y  BaseAlignAxisB=+Z  RotationStandardAxis=+Z  RotationAngle=-90  RotationAngleUnits=deg  RotationArbitraryAxis=[0 0 1]  RotationSequenceAxes=FollowerAxes  RotationSequence=XYX  RotationSequenceAngles=[0 0 0]  RotationSequenceAnglesUnits=deg  RotationMatrix=[1 0 0; 0 1 0; 0 0 1]  Quaternion=[1 0 0 0]  TranslationMethod=Cartesian  TranslationCartesianOffset=[0 0 0.7]  TranslationCartesianOffsetUnits=m  TranslationStandardAxis=+Z  TranslationStandardOffset=0  TranslationStandardOffsetUnits=m  TranslationROffset=0  TranslationROffsetUnits=m  TranslationThetaOffset=0  TranslationThetaOffsetUnits=deg  TranslationZOffset=0  TranslationZOffsetUnits=m
  Transform Neck : sm_lib/Frames and Transforms/Rigid Transform  RotationMethod=StandardAxis  FollAlignAxisA=+X  BaseAlignAxisA=+Y  FollAlignAxisB=+Y  BaseAlignAxisB=+Z  RotationStandardAxis=+X  RotationAngle=90  RotationAngleUnits=deg  RotationArbitraryAxis=[0 0 1]  RotationSequenceAxes=FollowerAxes  RotationSequence=XYX  RotationSequenceAngles=[0 0 0]  RotationSequenceAnglesUnits=deg  RotationMatrix=[1 0 0; 0 1 0; 0 0 1]  Quaternion=[1 0 0 0]  TranslationMethod=None  TranslationCartesianOffset=[0 0 0]  TranslationCartesianOffsetUnits=m  TranslationStandardAxis=+Z  TranslationStandardOffset=0  TranslationStandardOffsetUnits=m  TranslationROffset=0  TranslationROffsetUnits=m  TranslationThetaOffset=0  TranslationThetaOffsetUnits=deg  TranslationZOffset=0  TranslationZOffsetUnits=m
  F : PMIOPort  Side=Left
  C : PMIOPort  Port=2  Side=Right
  connections:
  Transform/RConn1 -- Transform Neck/LConn1
  Transform Neck/RConn1 -- F/RConn1
  Solid/RConn1 -- ReferenceFrame/RConn1 -- Transform/LConn1 -- Transform Head Center/LConn1
  C/RConn1 -- Transform Head Center/RConn1

== system Linkage/Susp/Linkage Decoupled/Steer/Rack Static Shafts/Driver/Human/Leg L ==
  Foot L : Subsystem
  Leg Lower L : Subsystem
  Leg Upper L : Subsystem
  Toe L : Subsystem
  P : PMIOPort  Side=Left
  connections:
  Leg Lower L/LConn2 -- Leg Upper L/LConn2
  Foot L/LConn1 -- Toe L/LConn1
  Leg Upper L/LConn1 -- P/RConn1
  Leg Lower L/LConn1 -- Foot L/LConn2

== system Linkage/Susp/Linkage Decoupled/Steer/Rack Static Shafts/Driver/Human/Leg R ==
  Foot R : Subsystem
  Leg Lower R : Subsystem
  Leg Upper R : Subsystem
  Toe R : Subsystem
  P : PMIOPort  Side=Left
  connections:
  Foot R/LConn1 -- Toe R/LConn1
  Leg Lower R/LConn2 -- Leg Upper R/LConn1
  P/RConn1 -- Leg Upper R/LConn2
  Leg Lower R/LConn1 -- Foot R/LConn2

== system Linkage/Susp/Linkage Decoupled/Steer/Rack Static Shafts/Driver/Human/Pelvis ==
  ReferenceFrame : sm_lib/Frames and Transforms/Reference Frame
  Solid : sm_lib/Body Elements/File Solid  ExtGeomFileName=Human_pelvis.STEP  UnitType=FromFile  ExtGeomFileUnits=m  StepReaderType=HEX  ExportConvexHullGeometry=off  InertiaType=CalculateFromGeometry  BasedOnType=Density  Density=rho_human  DensityUnits=kg/m^3  Mass=0  MassUnits=kg  CenterOfMass=[0 0 0]  CenterOfMassUnits=cm  MomentsOfInertia=[1 1 1]  MomentsOfInertiaUnits=kg*cm^2  ProductsOfInertia=[0 0 0]  ProductsOfInertiaUnits=kg*cm^2  GraphicType=FromGeometry  MarkerShape=Sphere  MarkerSize=10  GraphicVisPropType=SimpleVisualProperties  GraphicDiffuseColor=clr_human  GraphicOpacity=opc_human  GraphicSpecularColor=[0.5 0.5 0.5 1.0]  GraphicAmbientColor=[0.15 0.15 0.15 1.0]  GraphicEmissiveColor=[0.0 0.0 0.0 1.0]  GraphicShininess=75  DoExposeReferenceFrame=on  SerializedFrames=<Frames/>
  Transform : sm_lib/Frames and Transforms/Rigid Transform  RotationMethod=ArbitraryAxis  FollAlignAxisA=+X  BaseAlignAxisA=+Y  FollAlignAxisB=+Y  BaseAlignAxisB=+Z  RotationStandardAxis=+Z  RotationAngle=0  RotationAngleUnits=rad  RotationArbitraryAxis=[0 0 0]  RotationSequenceAxes=FollowerAxes  RotationSequence=XYX  RotationSequenceAngles=[0 0 0]  RotationSequenceAnglesUnits=deg  RotationMatrix=[1 0 0; 0 1 0; 0 0 1]  Quaternion=[1 0 0 0]  TranslationMethod=Cartesian  TranslationCartesianOffset=[-134.08000755 1.1899999995818e-06 -27.77000427]  TranslationCartesianOffsetUnits=mm  TranslationStandardAxis=+Z  TranslationStandardOffset=0  TranslationStandardOffsetUnits=mm  TranslationROffset=0  TranslationROffsetUnits=m  TranslationThetaOffset=0  TranslationThetaOffsetUnits=deg  TranslationZOffset=0  TranslationZOffsetUnits=m
  Transform2 : sm_lib/Frames and Transforms/Rigid Transform  RotationMethod=ArbitraryAxis  FollAlignAxisA=+X  BaseAlignAxisA=+Y  FollAlignAxisB=+Y  BaseAlignAxisB=+Z  RotationStandardAxis=+Z  RotationAngle=2.0943951023932  RotationAngleUnits=rad  RotationArbitraryAxis=[-0.577350269189626 -0.577350269189626 -0.577350269189626]  RotationSequenceAxes=FollowerAxes  RotationSequence=XYX  RotationSequenceAngles=[0 0 0]  RotationSequenceAnglesUnits=deg  RotationMatrix=[1 0 0; 0 1 0; 0 0 1]  Quaternion=[1 0 0 0]  TranslationMethod=Cartesian  TranslationCartesianOffset=[0 0 0]  TranslationCartesianOffsetUnits=mm  TranslationStandardAxis=+Z  TranslationStandardOffset=0  TranslationStandardOffsetUnits=mm  TranslationROffset=0  TranslationROffsetUnits=m  TranslationThetaOffset=0  TranslationThetaOffsetUnits=deg  TranslationZOffset=0  TranslationZOffsetUnits=m
  Transform3 : sm_lib/Frames and Transforms/Rigid Transform  RotationMethod=ArbitraryAxis  FollAlignAxisA=+X  BaseAlignAxisA=+Y  FollAlignAxisB=+Y  BaseAlignAxisB=+Z  RotationStandardAxis=+Z  RotationAngle=0.673691865560248  RotationAngleUnits=rad  RotationArbitraryAxis=[-0.990464172106651 0.133137430769094 0.0354280722209296]  RotationSequenceAxes=FollowerAxes  RotationSequence=XYX  RotationSequenceAngles=[0 0 0]  RotationSequenceAnglesUnits=deg  RotationMatrix=[1 0 0; 0 1 0; 0 0 1]  Quaternion=[1 0 0 0]  TranslationMethod=Cartesian  TranslationCartesianOffset=[25.5543445465301 17.9334803765627 4.01854756989799]  TranslationCartesianOffsetUnits=mm  TranslationStandardAxis=+Z  TranslationStandardOffset=0  TranslationStandardOffsetUnits=mm  TranslationROffset=0  TranslationROffsetUnits=m  TranslationThetaOffset=0  TranslationThetaOffsetUnits=deg  TranslationZOffset=0  TranslationZOffsetUnits=m
  Torso : PMIOPort  Side=Left
  LegL : PMIOPort  Port=2  Side=Right
  LegR : PMIOPort  Port=3  Side=Right
  connections:
  Transform3/RConn1 -- LegL/RConn1
  Transform2/RConn1 -- Torso/RConn1
  Transform/RConn1 -- LegR/RConn1
  Transform/LConn1 -- Transform2/LConn1 -- Transform3/LConn1 -- Solid/RConn1 -- ReferenceFrame/RConn1
